simulink model "model_ColumnSetup_00_pre_fable_mux_runtime_retry_20260703_051745"  (R2020b)
settings: Solver=ode4  StartTime=0.0  StopTime=tend  FixedStep=dt  RelTol=1e-3  EnableMultiTasking=on
model workspace (MAT data in the model file):
  controller_enable_switch = Simulink.Parameter
  controller_enable_switch.Value = 0
  controller_enable_switch.DataType = 'boolean'
  controller_enable_switch.Dimensions = [1 1]
  dd_pause_enable = Simulink.Parameter
  dd_pause_enable.Value = 1
  dd_pause_enable.Description = 'Dashboard flag for pausing time-history and sine command generation.'
  dd_pause_enable.DataType = 'auto'
  dd_pause_enable.Dimensions = [1 1]
  osi_gain_enable_initial = Simulink.Parameter
  osi_gain_enable_initial.Value = 0
  osi_gain_enable_initial.DataType = 'auto'
  osi_gain_enable_initial.Dimensions = [1 1]
  smooth_stop_enable = Simulink.Parameter
  smooth_stop_enable.Value = 1
  smooth_stop_enable.Description = 'Dashboard flag for smooth stop and smooth resume of the command.'
  smooth_stop_enable.DataType = 'auto'
  smooth_stop_enable.Dimensions = [1 1]
  zero_meas_enable = Simulink.Parameter
  zero_meas_enable.Value = 0
  zero_meas_enable.Description = 'Dashboard flag for actuator-on adaptive command trim that drives measured displacement back to zero.'
  zero_meas_enable.DataType = 'auto'
  zero_meas_enable.Dimensions = [1 1]
undefined symbols (not defined in the file or in its folder): amp_2_percentile, blwnStdFromExceedance, command_channel_selector, correction_gain, dt, exceed_percentile, f1, f_final, f_init, fbla, fblag, fblbins, fblfbins, fblfw, fbls, fblw, hs_ag, hs_C, hs_force_sign_codegen, hs_force_to_floor, hs_ground_force_gain, hs_interface_from_floor, hs_interface_from_force, hs_K, hs_M, hs_time, hs_time_scale_factor_codegen, phase_lead_den, phase_lead_num, sat_limit, t_ending, tend_chirp, time_history, v2a_gain, v2d_gain, v2f_gain, zero_alpha
libraries: simulink x2, speedgoatlib_IO113 x2, speedgoatlib_IO112 x2, dsparch4 x1, slrealtimeloglib x1, slpidlib x1
settings Model: SimulationMode=external  ExtModeEnableFloating=off  OrderedModelArguments=off  Creator=User  LastModifiedBy=BOWN1111PC1
settings SolverCC: ConcurrentTasks=on  PositivePriorityOrder=on
settings DataIOCC: LimitDataPoints=on  SaveFormat=Array  ReturnWorkspaceOutputs=off
settings OptimizationCC: BlockReduction=off  OptimizeBlockIOStorage=off  BufferReuse=off  ExpressionFolding=off  LocalBlockOutputs=off
settings DebuggingCC: UnderspecifiedInitializationDetection=Classic  MergeDetectMultiDrivingBlocksExec=none  SolverPrmCheckMsg=warning  TasksWithSamePriorityMsg=none  StateNameClashWarn=warning  SFUnexpectedBacktrackingDiag=warning  SFNoUnconditionalDefaultTransitionDiag=warning  SFExecutionAtInitializationDiag=none  ArithmeticOperatorsInVariantConditions=warning
settings HardwareCC: ProdBitPerLong=64  ProdLongLongMode=on  ProdHWDeviceType=Intel->x86-64 (Linux 64)
settings ModelReferenceCC: PropagateSignalLabelsOutOfModel=off
settings SFSimCC: SimUseLocalCustomCode=off  CustomCodeUndefinedFunction=UseInterfaceOnly
settings RTWCC: Description=Simulink Real-Time  SystemTargetFile=slrealtime.tlc  TemplateMakefile=slrealtime_default_tmf  RTWVerbose=off  RTWUseLocalCustomCode=off  Toolchain=Simulink Real-Time Toolchain  BuildConfiguration=Faster Runs  CodeExecutionProfiling=on  TargetLang=C++
settings CodeAppCC: StateflowObjectComments=on
settings ConfigComp: CovMetricSettings=dw  CovSaveCumulativeToWorkspaceVar=on  CovSaveSingleToWorkspaceVar=on  CovExternalEMLEnable=off

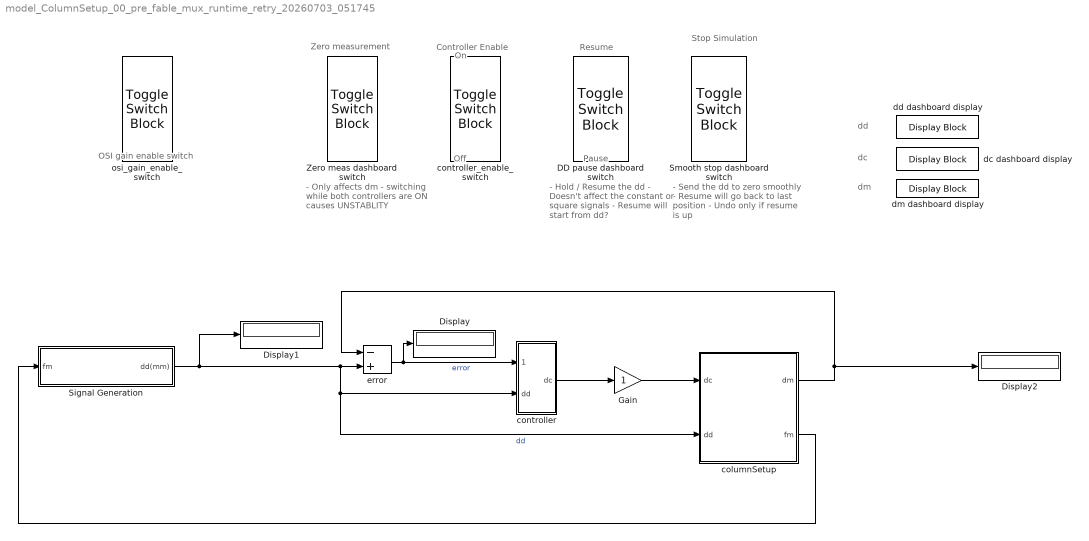
== system model_ColumnSetup_00_pre_fable_mux_runtime_retry_20260703_051745 ==
  note: Pause
  note: Resume
  note: Stop Simulation
  note: - Send the dd to zero smoothly
      | - Resume will go back to last position
      | - Undo only if resume is up
  note: Zero measurement
  note: - Hold / Resume the dd
      | - Doesn't affect the constant or square signals
      | - Resume will start from dd?
  note: - Only affects dm
      | - switching while both controllers are ON causes UNSTABLITY
  note: dd
  note: dc
  note: dm
  note: Controller Enable
  note: On
  note: Off
  note: OSI gain enable switch
  DD pause dashboard switch : ToggleSwitchBlock  LabelPosition=Hide
      settings: Values={{'Zero', ''}, [1 0]}
  Display : Display
      settings: SampleTime=dt
  Display1 : Display
      settings: SampleTime=dt
  Display2 : Display
      settings: SampleTime=dt
  Gain : Gain
  Signal Generation : Subsystem
  Smooth stop dashboard switch : ToggleSwitchBlock  LabelPosition=Hide
      settings: Values={{'Zero', ''}, [0 1]}
  Zero meas dashboard switch : ToggleSwitchBlock  LabelPosition=Hide
      settings: Values={{'Zero', ''}, [0 1]}
  columnSetup : Subsystem
  controller : Subsystem
  controller_enable_switch : ToggleSwitchBlock  LabelPosition=Hide
      settings: Values={{'zero', ''}, [0 1]}
  dc dashboard display : DisplayBlock  LabelPosition=Hide  Format=Custom  Transparency=1  FormatString=%.3f
  dd dashboard display : DisplayBlock  LabelPosition=Hide  Format=Custom  Transparency=1  FormatString=%.3f
  dm dashboard display : DisplayBlock  LabelPosition=Hide  Format=Custom  Transparency=1  FormatString=%.3f
  error : Sum  Inputs=-+  SampleTime=dt
  osi_gain_enable_switch : ToggleSwitchBlock  LabelPosition=Hide
      settings: Values={{'zero', ''}, [0 1]}
  wires:
  columnSetup/1(dm) -> error/1, Display2/1
  error/1 -> Display/1, controller/1(error)  "error"
  controller/1(dc) -> Gain/1
  Signal Generation/1(dd(mm)) -> columnSetup/2(dd), controller/2(dd), error/2, Display1/1  "dd"
  columnSetup/2(fm) -> Signal Generation/1(fm)
  Gain/1 -> columnSetup/1(dc)

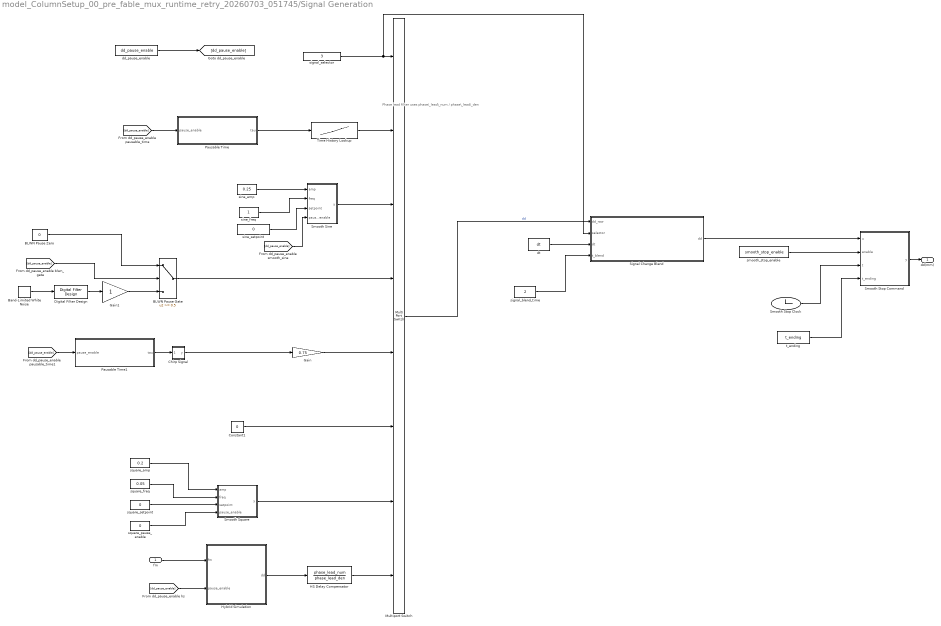
== system model_ColumnSetup_00_pre_fable_mux_runtime_retry_20260703_051745/Signal Generation ==
  note: Phase lead filter uses phase\_lead\_num / phase\_lead\_den
  fm : Inport
  BLWN Pause Gate : Switch  Threshold=0.5  SampleTime=dt
  BLWN Pause Zero : Constant  Value=0  SampleTime=dt
  Band-Limited White Noise : simulink/Sources/Band-Limited White Noise  Cov=blwnStdFromExceedance(amp_2_percentile, exceed_percentile)^2*dt/sum((fir1(130, 2*f1*dt)).^2)  Ts=dt  seed=[22451]
  Chirp Signal : Subsystem  AncestorBlock=simulink/Sources/Chirp Signal  mask(chirp){f1=f_init, T=tend_chirp, f2=f_final, VectorParams1D=on}
      mask prompts: f1 "Simulink:masks:InitialFrequencyHz_MP"; T "Simulink:masks:TargetTimesecs_MP"; f2 "Simulink:masks:FrequencyAtTargetTimeHz_MP"; VectorParams1D "Simulink:masks:InterpretVectorParametersAs1D_MP"
      mask help: Simulink:masks:chirp_MD
      mask init:
      | blkName = gcb;
      | t=[0:.1:5];
      | set_param([blkName '/targetTime'], 'VectorParams1D', VectorParams1D);
      | set_param([blkName '/initialFreq'], 'VectorParams1D', VectorParams1D);
      | set_param([blkName '/deltaFreq'], 'VectorParams1D', VectorParams1D);
      mask Help: The chirp signal has linearly increasing frequency with time.  This block can be used for spectral analysis of nonlinear systems.
      mask Display: plot(t,sin(t.*t))
  Constant1 : Constant  Value=0  SampleTime=dt
  Digital Filter Design : dsparch4/Digital Filter Design  mwdsp_browser_bugfix_var=off
      link override Digital Filter: Coefficients=fir1(130, 2*f1*dt)
  Gain : Gain  Gain=0.75  SampleTime=dt
  Gain1 : Gain  SampleTime=dt
  HS Delay Compensator : DiscreteTransferFcn  Numerator=phase_lead_num  Denominator=phase_lead_den  SampleTime=dt
  Hybrid Simulation : MATLAB Function  TreatAsAtomicUnit=on
  Multiport Switch : MultiPortSwitch  Inputs=7  SampleTime=dt
  Pausable Time : MATLAB Function  TreatAsAtomicUnit=on
  Pausable Time1 : MATLAB Function  TreatAsAtomicUnit=on
  Signal Change Blend : MATLAB Function  TreatAsAtomicUnit=on
  Smooth Sine : MATLAB Function  TreatAsAtomicUnit=on
  Smooth Square : MATLAB Function  TreatAsAtomicUnit=on
  Smooth Stop Clock : Clock
  Smooth Stop Command : MATLAB Function  TreatAsAtomicUnit=on
  Time History Lookup : Lookup_n-D  NumberOfTableDimensions=1  BreakpointsForDimension1=time_history(:,1)  Table=time_history(:,2)  ExtrapMethod=Clip  SampleTime=dt  InternalRulePriority=Speed  RndMeth=Simplest  InputSameDT=on
  dd_pause_enable : Constant  Value=dd_pause_enable  SampleTime=dt
  dt : Constant  Value=dt  SampleTime=dt
  signal_blend_time : Constant  Value=2  SampleTime=dt
  signal_selector : Constant  Value=3  SampleTime=dt
  sine_amp : Constant  Value=0.25  SampleTime=dt
  sine_freq : Constant  SampleTime=dt
  sine_setpoint : Constant  Value=0  SampleTime=dt
  smooth_stop_enable : Constant  Value=smooth_stop_enable  SampleTime=dt
  square_amp : Constant  Value=0.2  SampleTime=dt
  square_freq : Constant  Value=0.05  SampleTime=dt
  square_pause_enable : Constant  Value=0  SampleTime=dt
  square_setpoint : Constant  Value=0  SampleTime=dt
  t_ending : Constant  Value=t_ending  SampleTime=dt
  dd(mm) : Outport  SampleTime=dt
  wires:
  signal_selector/1 -> Signal Change Blend/2(selector), Multiport Switch/1
  Chirp Signal/1(y) -> Gain/1
  Smooth Sine/1(y) -> Multiport Switch/3
  Band-Limited White Noise/1 -> Digital Filter Design/1
  Digital Filter Design/1 -> Gain1/1
  Gain/1 -> Multiport Switch/5
  Constant1/1 -> Multiport Switch/6
  Pausable Time/1(tau) -> Time History Lookup/1
  Time History Lookup/1 -> Multiport Switch/2
  BLWN Pause Zero/1 -> BLWN Pause Gate/1
  Gain1/1 -> BLWN Pause Gate/3
  BLWN Pause Gate/1 -> Multiport Switch/4
  [dd_pause_enable] -> Pausable Time/1(pause_enable)
  [dd_pause_enable] -> BLWN Pause Gate/2
  Pausable Time1/1(tau) -> Chirp Signal/1(tau)
  [dd_pause_enable] -> Pausable Time1/1(pause_enable)
  sine_amp/1 -> Smooth Sine/1(amp)
  sine_freq/1 -> Smooth Sine/2(freq)
  sine_setpoint/1 -> Smooth Sine/3(setpoint)
  [dd_pause_enable] -> Smooth Sine/4(pause_enable)
  smooth_stop_enable/1 -> Smooth Stop Command/2(enable)
  Smooth Stop Clock/1 -> Smooth Stop Command/3(t)
  t_ending/1 -> Smooth Stop Command/4(t_ending)
  dt/1 -> Signal Change Blend/3(dt)
  signal_blend_time/1 -> Signal Change Blend/4(t_blend)
  Multiport Switch/1 -> Signal Change Blend/1(dd_raw)  "dd"
  Signal Change Blend/1(dd) -> Smooth Stop Command/1(u)
  square_amp/1 -> Smooth Square/1(amp)
  square_freq/1 -> Smooth Square/2(freq)
  square_setpoint/1 -> Smooth Square/3(setpoint)
  square_pause_enable/1 -> Smooth Square/4(pause_enable)
  Smooth Square/1(y) -> Multiport Switch/7
  Smooth Stop Command/1(y) -> dd(mm)/1
  dd_pause_enable/1 -> [dd_pause_enable]
  fm/1 -> Hybrid Simulation/1(fm)
  [dd_pause_enable] -> Hybrid Simulation/2(pause_enable)
  Hybrid Simulation/1(dd) -> HS Delay Compensator/1
  HS Delay Compensator/1 -> Multiport Switch/8

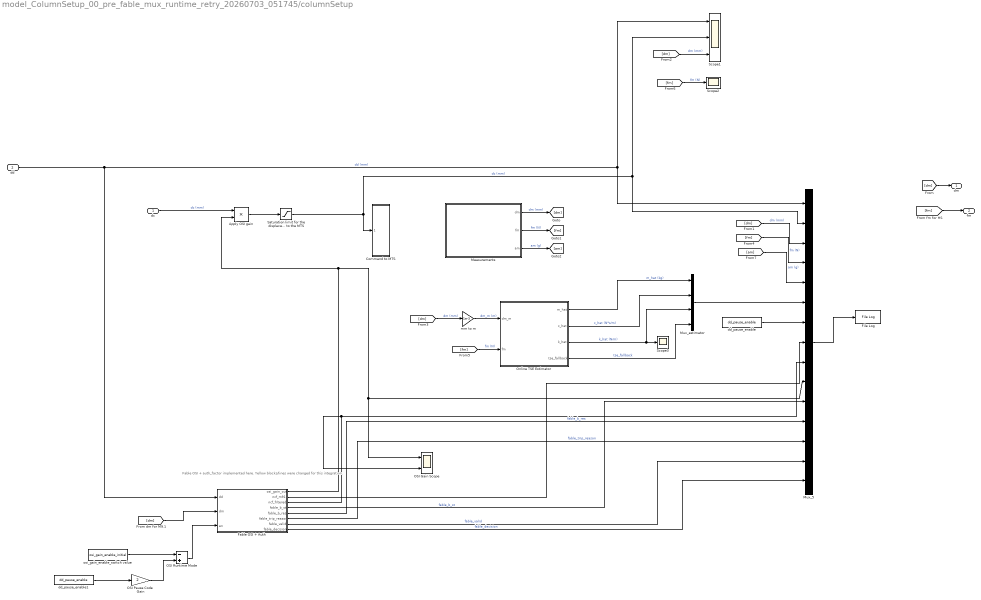
== system model_ColumnSetup_00_pre_fable_mux_runtime_retry_20260703_051745/columnSetup ==
  note: Fable OSI + auth_factor implemented here. Yellow blocks/lines were changed for this integration.
  dc : Inport  SampleTime=dt
  dd : Inport  Port=2  SampleTime=dt
  Apply OSI gain : Product  Inputs=**
  Command to MTS : Subsystem
  Fable OSI + Auth : MATLAB Function  TreatAsAtomicUnit=on
  File Log : slrealtimeloglib/File Log  decimation=1
      settings: SourceProductBaseCode=XP
  Measurements : Subsystem
  Mux_5 : Mux  Inputs=15
  Mux_estimator : Mux
  OSI Gain Scope : Scope  NumInputPorts=2
  OSI Pause Code Gain : Gain  Gain=2
  OSI Runtime Mode : Sum  Inputs=-+  SampleTime=dt
  Online TSE Estimator : MATLAB Function  TreatAsAtomicUnit=on
  Saturation limit for the displacement signal that is sent to the MTS : Saturate  UpperLimit=sat_limit  LowerLimit=-sat_limit  SampleTime=dt
  Scope1 : Scope  NumInputPorts=3
  Scope2 : Scope
  Scope3 : Scope
  dd_pause_enable : Constant  Value=dd_pause_enable  SampleTime=dt
  dd_pause_enable1 : Constant  Value=dd_pause_enable  SampleTime=dt
  mm to m : Gain  Gain=1e-3
  osi_gain_enable_switch value : Constant  Value=osi_gain_enable_initial
  dm : Outport  SampleTime=dt
  fm : Outport  Port=2  SampleTime=dt
  wires:
  Saturation limit for the displacement signal that is sent to the MTS/1 -> Mux_5/2, Scope1/2, Command to MTS/1(dc (mm))  "dc (mm)"
  Mux_5/1 -> File Log/1
  Measurements/1(dm) -> [dm]  "dm (mm)"
  [am] -> Mux_5/5  "am (g)"
  dd/1 -> Mux_5/1, Scope1/1, Fable OSI + Auth/1(dd)  "dd (mm)"
  Online TSE Estimator/1(m_hat) -> Mux_estimator/1  "m_hat (kg)"
  Online TSE Estimator/2(c_hat) -> Mux_estimator/2  "c_hat (N*s/m)"
  Online TSE Estimator/3(k_hat) -> Scope3/1, Mux_estimator/3  "k_hat (N/m)"
  Online TSE Estimator/4(tse_fallback) -> Mux_estimator/4  "tse_fallback"
  [dm] -> dm/1
  [dm] -> Mux_5/3  "dm (mm)"
  [dm] -> Scope1/3  "dm (mm)"
  Measurements/2(fm) -> [fm]  "fm (N)"
  [fm] -> Mux_5/4  "fm (N)"
  [fm] -> Online TSE Estimator/2(fm)  "fm (N)"
  [fm] -> Scope2/1  "fm (N)"
  Measurements/3(am) -> [am]  "am (g)"
  Mux_estimator/1 -> Mux_5/6
  [dm] -> mm to m/1  "dm (mm)"
  mm to m/1 -> Online TSE Estimator/1(dm_m)  "dm_m (m)"
  [fm] -> fm/1
  dd_pause_enable/1 -> Mux_5/7
  dc/1 -> Apply OSI gain/1  "dc (mm)"
  Apply OSI gain/1 -> Saturation limit for the displacement signal that is sent to the MTS/1
  osi_gain_enable_switch value/1 -> OSI Runtime Mode/1
  Fable OSI + Auth/1(osi_gain_out) -> Apply OSI gain/2, OSI Gain Scope/1, Mux_5/10
  Fable OSI + Auth/3(ncf_filtered) -> OSI Gain Scope/2, Mux_5/9
  Fable OSI + Auth/2(ncf_m91) -> Mux_5/8
  [dm] -> Fable OSI + Auth/2(dm)
  OSI Pause Code Gain/1 -> OSI Runtime Mode/2
  OSI Runtime Mode/1 -> Fable OSI + Auth/3(en)
  Fable OSI + Auth/4(fable_b_st) -> Mux_5/11  "fable_b_st"
  Fable OSI + Auth/5(fable_b_res) -> Mux_5/12  "fable_b_res"
  Fable OSI + Auth/6(fable_trip_reason) -> Mux_5/13  "fable_trip_reason"
  Fable OSI + Auth/7(fable_valid) -> Mux_5/14  "fable_valid"
  Fable OSI + Auth/8(fable_decision) -> Mux_5/15  "fable_decision"
  dd_pause_enable1/1 -> OSI Pause Code Gain/1

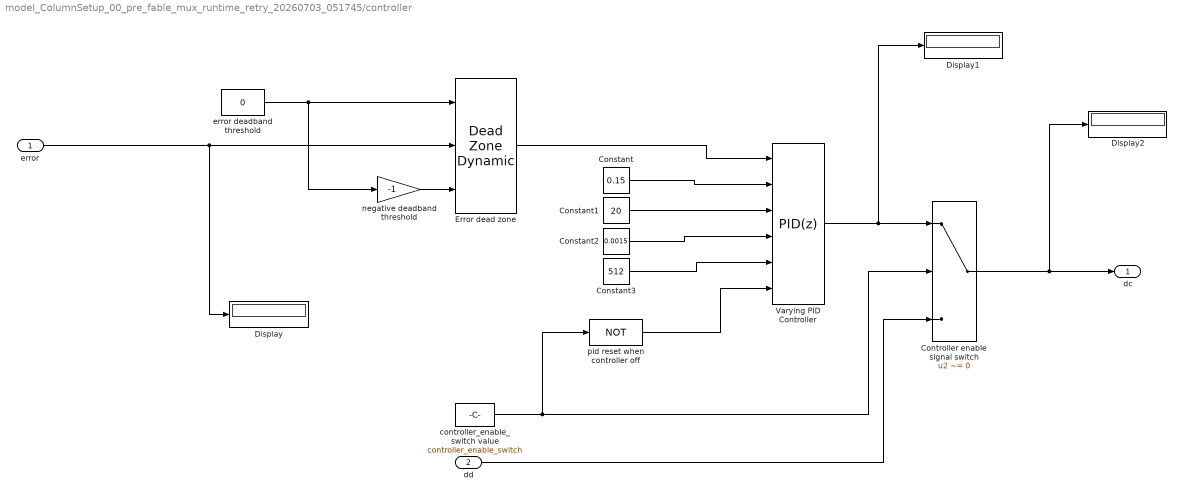
== system model_ColumnSetup_00_pre_fable_mux_runtime_retry_20260703_051745/controller ==
  error : Inport  SampleTime=dt
  dd : Inport  Port=2  SampleTime=dt
  Constant : Constant  Value=0.15  SampleTime=dt
  Constant1 : Constant  Value=20  SampleTime=dt
  Constant2 : Constant  Value=0.0015  SampleTime=dt
  Constant3 : Constant  Value=512  SampleTime=dt
  Controller enable signal switch : Switch  Criteria=u2 ~= 0  SampleTime=dt
  Display : Display
      settings: SampleTime=dt
  Display1 : Display
      settings: SampleTime=dt
  Display2 : Display
      settings: SampleTime=dt
  Error dead zone : simulink/Discontinuities/Dead Zone Dynamic
      settings: SourceProductBaseCode=SL
  Varying PID Controller : slpidlib/PID Controller  Controller=PID  Form=Parallel  TimeDomain=Discrete-time  UseExternalTs=off  SampleTime=dt  IntegratorMethod=Forward Euler  FilterMethod=Forward Euler  ControllerParametersSource=external  P=1  I=1  D=0  UseFilter=on  N=100  TunerSelectOption=Transfer Function Based (PID Tuner App)  InitialConditionSource=internal  InitialConditionForIntegrator=0  InitialConditionForFilter=0  DifferentiatorICPrevScaledInput=0  ExternalReset=level  TrackingMode=off  Kt=1  LimitOutput=off  SatLimitsSource=internal  UpperSaturationLimit=inf  LowerSaturationLimit=-inf  LinearizeAsGain=on  AntiWindupMode=none  Kb=1  POutMin=[]  POutMax=[]  IOutMin=[]  IOutMax=[]  DOutMin=[]  DOutMax=[]  NOutMin=[]  NOutMax=[]  SumOutMin=[]  SumOutMax=[]  SaturationOutMin=[]  SaturationOutMax=[]  PParamMin=[]  PParamMax=[]  IParamMin=[]  IParamMax=[]  DParamMin=[]  DParamMax=[]  NParamMin=[]  NParamMax=[]  KbParamMin=[]  KbParamMax=[]  KtParamMin=[]  KtParamMax=[]  KbOutMin=[]  KbOutMax=[]  KtOutMin=[]  KtOutMax=[]  IntegratorOutMin=[]  IntegratorOutMax=[]  FilterOutMin=[]  FilterOutMax=[]  SumI1OutMin=[]  SumI1OutMax=[]  SumI2OutMin=[]  SumI2OutMax=[]  SumI3OutMin=[]  SumI3OutMax=[]  SumI4OutMin=[]  SumI4OutMax=[]  SumDOutMin=[]  SumDOutMax=[]  DifferentiatorOutMin=[]  DifferentiatorOutMax=[]  FilterDiffOutCoefMin=[]  FilterDiffOutCoefMax=[]  ReciprocalOutMin=[]  ReciprocalOutMax=[]  SumDenOutMin=[]  SumDenOutMax=[]  SumNumOutMin=[]  SumNumOutMax=[]  DivideOutMin=[]  DivideOutMax=[]  UdiffTsProdOutMin=[]  UdiffTsProdOutMax=[]  NTsProdOutMin=[]  NTsProdOutMax=[]  UintegralTsProdOutMin=[]  UintegralTsProdOutMax=[]  UngainTsProdOutMin=[]  UngainTsProdOutMax=[]  IntegratorContinuousStateAttributes=''  IntegratorStateMustResolveToSignalObject=off  IntegratorRTWStateStorageClass=Auto  FilterContinuousStateAttributes=''  FilterStateMustResolveToSignalObject=off  FilterRTWStateStorageClass=Auto  ParallelPVariant=ExternalParameters  IdealPVariant=Disabled  IVariant=ExternalParameters  DVariant=ExternalParameters  IntegratorVariant=Discrete  SatVariant=Disabled  AWVariant=Passthrough  PCopyVariant=Disabled  TRVariant=Disabled  FdbkBlocksVariant=Forward  IdealPFdbkVariant=Disabled  SatFdbkVariant=Disabled  DerivativeFilterVariant=ForwardEulerFilter  NVariant=ExternalParameters  NCopyVariant=Disabled  FilterICVariant=InternalICsFilter  IntegratorICVariant=InternalICs  ExternalResetVariant=ExternalReset  TRSumVariant=Passthrough  SumFdbkVariant=Disabled  SumVariant=Sum_PID  TsampFilterVariant=InternalTs  TsampNgainVariant=Passthrough  TsampIntegralVariant=Passthrough  ExternalSaturationOutDataTypeStr=Inherit: Same as second input
  controller_enable_switch value : Constant  Value=controller_enable_switch  OutDataTypeStr=boolean  SampleTime=dt
  error deadband threshold : Constant  Value=0
  negative deadband threshold : Gain  Gain=-1
  pid reset when controller off : Logic  Operator=NOT  AllPortsSameDT=off  OutDataTypeStr=boolean
  dc : Outport  SampleTime=dt
  wires:
  error/1 -> Error dead zone/2, Display/1
  controller_enable_switch value/1 -> Controller enable signal switch/2, pid reset when controller off/1
  Controller enable signal switch/1 -> Display2/1, dc/1
  Constant3/1 -> Varying PID Controller/5
  Constant1/1 -> Varying PID Controller/3
  dd/1 -> Controller enable signal switch/3
  Constant2/1 -> Varying PID Controller/4
  Constant/1 -> Varying PID Controller/2
  Varying PID Controller/1 -> Display1/1, Controller enable signal switch/1
  pid reset when controller off/1 -> Varying PID Controller/6
  error deadband threshold/1 -> negative deadband threshold/1, Error dead zone/1
  negative deadband threshold/1 -> Error dead zone/3
  Error dead zone/1 -> Varying PID Controller/1

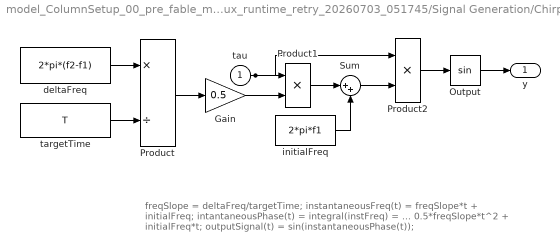
== system model_ColumnSetup_00_pre_fable_mux_runtime_retry_20260703_051745/Signal Generation/Chirp Signal ==
  note: freqSlope = deltaFreq/targetTime;
      | instantaneousFreq(t) = freqSlope*t + initialFreq;
      | intantaneousPhase(t) = integral(instFreq) = ...
      |       0.5*freqSlope*t^2 + initialFreq*t;
      | outputSignal(t) = sin(instantaneousPhase(t));
  tau : Inport
  Gain : Gain  DisableCoverage=on  Gain=0.5  OutDataTypeStr=Inherit: Same as input  ParamDataTypeStr=Inherit: Same as input
  Output : Trigonometry
  Product : Product  DisableCoverage=on  Inputs=*/  InputSameDT=on  SaturateOnIntegerOverflow=on  OutDataTypeStr=Inherit: Same as first input
  Product1 : Product  DisableCoverage=on  InputSameDT=on  SaturateOnIntegerOverflow=on  OutDataTypeStr=Inherit: Same as first input
  Product2 : Product  DisableCoverage=on  InputSameDT=on  SaturateOnIntegerOverflow=on  OutDataTypeStr=Inherit: Same as first input
  Sum : Sum  DisableCoverage=on  Inputs=|++  InputSameDT=on  SaturateOnIntegerOverflow=on  OutDataTypeStr=Inherit: Same as first input
  deltaFreq : Constant  DisableCoverage=on  Value=2*pi*(f2-f1)
  initialFreq : Constant  DisableCoverage=on  Value=2*pi*f1
  targetTime : Constant  DisableCoverage=on  Value=T
  y : Outport
  wires:
  Output/1 -> y/1
  Product2/1 -> Output/1
  Sum/1 -> Product2/2
  initialFreq/1 -> Sum/2
  Product1/1 -> Sum/1
  Gain/1 -> Product1/2
  Product/1 -> Gain/1
  targetTime/1 -> Product/2
  deltaFreq/1 -> Product/1
  tau/1 -> Product2/1, Product1/1

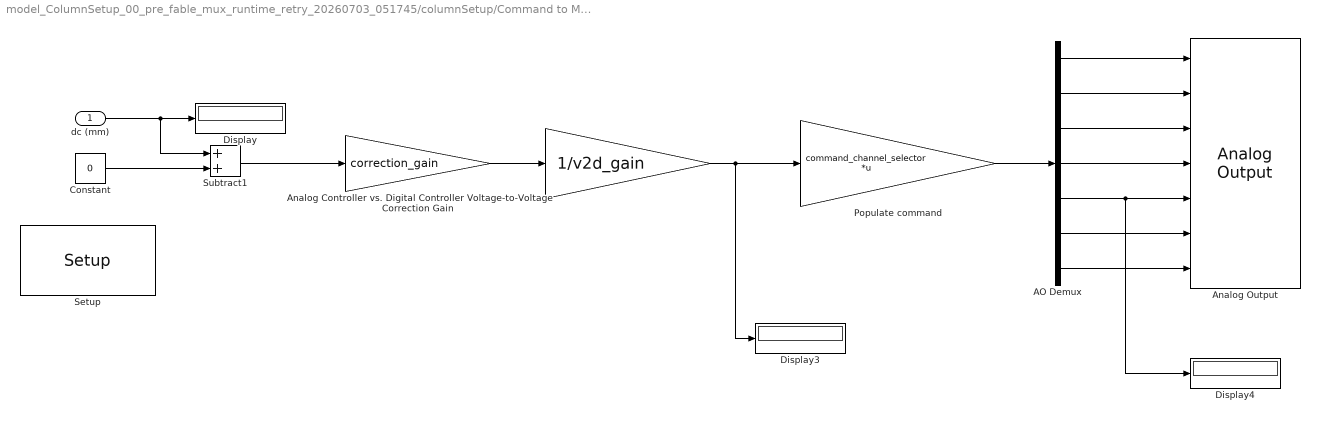
== system model_ColumnSetup_00_pre_fable_mux_runtime_retry_20260703_051745/columnSetup/Command to MTS ==
  dc (mm) : Inport  SampleTime=dt
  "  " : Gain  Gain=1/v2d_gain  SampleTime=dt
  " Analog Controller vs. Digital Controller Voltage-to-Voltage Correction Gain  " : Gain  Gain=correction_gain  SampleTime=dt
  AO Demux : Demux  Outputs=7
  Analog Output : speedgoatlib_IO113/Analog Output  id=1  index=[1,2,3,4,5,6,7]  channels=[1,2,3,4,5,6,7]  range=1  ts=dt  pciSlot=-1
      settings: SourceProductName=Simulink Real-Time: Speedgoat I/O Blockset
  Constant : Constant  Value=0  SampleTime=dt
  Display : Display
      settings: SampleTime=dt
  Display3 : Display
      settings: SampleTime=dt
  Display4 : Display
      settings: SampleTime=dt
  Populate command : Gain  Gain=command_channel_selector  Multiplication=Matrix(K*u)  SampleTime=dt
  Setup : speedgoatlib_IO113/Setup  group=Analog output setup  id=1  range=+-10V  daMode=Differential  triggerSignal=TTL  cal=off  dioDirLo=Output  dioDirHi=Input  pciSlot=-1  daChannel=[1,2,3,4,5,6,7]  daInitValue=[0 0 0 0 0 0 0]  daReset=[0]  doChannel=[1,2,3,4]  diChannel=[5,6,7,8]  doInitValue=[0]  doReset=[1]
      settings: SourceProductName=Simulink Real-Time: Speedgoat I/O Blockset
  Subtract1 : Sum  SampleTime=dt
  wires:
  " Analog Controller vs. Digital Controller Voltage-to-Voltage Correction Gain  "/1 -> "  "/1
  AO Demux/6 -> Analog Output/6
  AO Demux/3 -> Analog Output/3
  AO Demux/1 -> Analog Output/1
  AO Demux/4 -> Analog Output/4
  AO Demux/2 -> Analog Output/2
  Constant/1 -> Subtract1/2
  AO Demux/7 -> Analog Output/7
  Populate command/1 -> AO Demux/1
  Subtract1/1 -> " Analog Controller vs. Digital Controller Voltage-to-Voltage Correction Gain  "/1
  "  "/1 -> Display3/1, Populate command/1
  dc (mm)/1 -> Subtract1/1, Display/1
  AO Demux/5 -> Display4/1, Analog Output/5

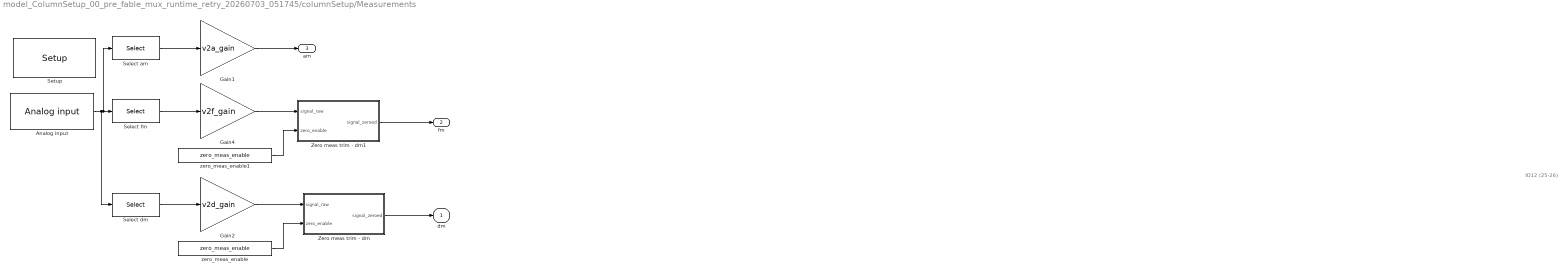
== system model_ColumnSetup_00_pre_fable_mux_runtime_retry_20260703_051745/columnSetup/Measurements ==
  note: IO12 (25-26)
  Analog input : speedgoatlib_IO112/Analog input  id=1  ts=dt  channels=18  range=1  resolution=1  pciSlot=-1
      settings: SourceProductName=Simulink Real-Time: Speedgoat I/O Blockset
  Gain1 : Gain  Gain=v2a_gain  SampleTime=dt
  Gain2 : Gain  Gain=v2d_gain  SampleTime=dt
  Gain4 : Gain  Gain=v2f_gain  SampleTime=dt
  Select am : Selector  InputPortWidth=18  SampleTime=dt  IndexOptions=Index vector (dialog)  Indices=ch.am  OutputSizes=1
  Select dm : Selector  InputPortWidth=18  SampleTime=dt  IndexOptions=Index vector (dialog)  Indices=ch.dm  OutputSizes=1
  Select fm : Selector  InputPortWidth=18  SampleTime=dt  IndexOptions=Index vector (dialog)  Indices=ch.fm  OutputSizes=1
  Setup : speedgoatlib_IO112/Setup  group=Analog input setup  id=1  cal=off  initiator=Initiator  invertIO=off  pciSlot=-1  adResolution=18bit (no data packing)  adChannel=18  adRange=+-10V  adCoupling=Differential
      settings: SourceProductName=Simulink Real-Time: Speedgoat I/O Blockset
  Zero meas trim - dm : Subsystem
  Zero meas trim - dm1 : Subsystem
  zero_meas_enable : Constant  Value=zero_meas_enable  SampleTime=dt
  zero_meas_enable1 : Constant  Value=zero_meas_enable  SampleTime=dt
  dm : Outport  SampleTime=dt
  fm : Outport  Port=2  SampleTime=dt
  am : Outport  Port=3  SampleTime=dt
  wires:
  Gain2/1 -> Zero meas trim - dm/1(signal_raw)
  Gain4/1 -> Zero meas trim - dm1/1(signal_raw)
  zero_meas_enable1/1 -> Zero meas trim - dm1/2(zero_enable)
  zero_meas_enable/1 -> Zero meas trim - dm/2(zero_enable)
  Zero meas trim - dm1/1(signal_zeroed) -> fm/1
  Zero meas trim - dm/1(signal_zeroed) -> dm/1
  Select dm/1 -> Gain2/1
  Select am/1 -> Gain1/1
  Select fm/1 -> Gain4/1
  Gain1/1 -> am/1
  Analog input/1 -> Select fm/1, Select am/1, Select dm/1

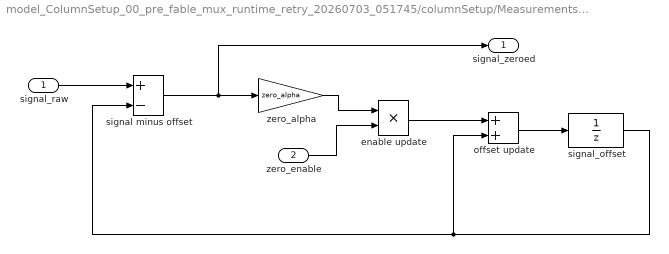
== system model_ColumnSetup_00_pre_fable_mux_runtime_retry_20260703_051745/columnSetup/Measurements/Zero meas trim - dm ==
  signal_raw : Inport  SampleTime=dt
  zero_enable : Inport  Port=2  SampleTime=dt
  enable update : Product  SampleTime=dt
  offset update : Sum  SampleTime=dt
  signal minus offset : Sum  Inputs=+-  SampleTime=dt
  signal_offset : UnitDelay  SampleTime=dt  HasFrameUpgradeWarning=on
  zero_alpha : Gain  Gain=zero_alpha  SampleTime=dt
  signal_zeroed : Outport  SampleTime=dt
  wires:
  offset update/1 -> signal_offset/1
  enable update/1 -> offset update/1
  zero_enable/1 -> enable update/2
  zero_alpha/1 -> enable update/1
  signal minus offset/1 -> zero_alpha/1, signal_zeroed/1
  signal_offset/1 -> signal minus offset/2, offset update/2
  signal_raw/1 -> signal minus offset/1

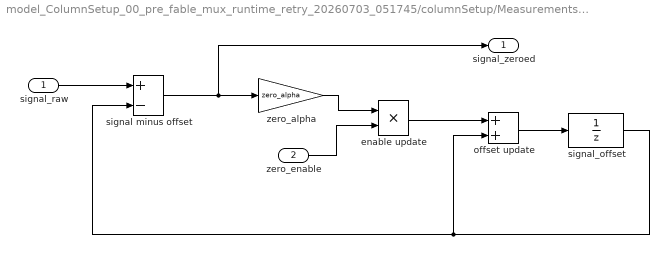
== system model_ColumnSetup_00_pre_fable_mux_runtime_retry_20260703_051745/columnSetup/Measurements/Zero meas trim - dm1 ==
  signal_raw : Inport  SampleTime=dt
  zero_enable : Inport  Port=2  SampleTime=dt
  enable update : Product  SampleTime=dt
  offset update : Sum  SampleTime=dt
  signal minus offset : Sum  Inputs=+-  SampleTime=dt
  signal_offset : UnitDelay  SampleTime=dt  HasFrameUpgradeWarning=on
  zero_alpha : Gain  Gain=zero_alpha  SampleTime=dt
  signal_zeroed : Outport  SampleTime=dt
  wires:
  offset update/1 -> signal_offset/1
  enable update/1 -> offset update/1
  zero_enable/1 -> enable update/2
  zero_alpha/1 -> enable update/1
  signal minus offset/1 -> zero_alpha/1, signal_zeroed/1
  signal_offset/1 -> signal minus offset/2, offset update/2
  signal_raw/1 -> signal minus offset/1

== matlab function model_ColumnSetup_00_pre_fable_mux_runtime_retry_20260703_051745/Signal Generation/Hybrid Simulation ==
  data: fm input; dd output; pause_enable input; hs_M parameter; hs_C parameter; hs_K parameter; hs_force_to_floor parameter; hs_interface_from_floor parameter; hs_interface_from_force parameter; hs_ground_force_gain parameter; hs_time parameter; hs_ag parameter; hs_time_scale_factor_codegen parameter; hs_force_sign_codegen parameter; dt parameter
function dd = hybrid_simulation(fm, pause_enable, hs_M, hs_C, hs_K, hs_force_to_floor, hs_interface_from_floor, hs_interface_from_force, hs_ground_force_gain, hs_time, hs_ag, hs_time_scale_factor_codegen, hs_force_sign_codegen, dt)
%#codegen
% WARNING - SAFETY CRITICAL: this block sends live HS command displacement.
% Keep force sign, interface equations, units, and stepping aligned with step_HS.m and num_exp.m.
persistent state
if isempty(state)
    state = zeros(12, 1);
end
cfg.n_floor = 3;
cfg.M = hs_M;
cfg.C = hs_C;
cfg.K = hs_K;
cfg.force_to_floor = hs_force_to_floor;
cfg.interface_from_floor = hs_interface_from_floor;
cfg.interface_from_force = hs_interface_from_force;
cfg.ground_force_gain = hs_ground_force_gain;
cfg.time = hs_time;
cfg.ag = hs_ag;
cfg.time_scale_factor = hs_time_scale_factor_codegen;
cfg.force_sign = hs_force_sign_codegen;
[dd, state] = step_HS(fm, pause_enable, dt, cfg, state);
end

== matlab function model_ColumnSetup_00_pre_fable_mux_runtime_retry_20260703_051745/columnSetup/Fable OSI + Auth ==
  data: dd input double size=1; osi_gain_out output double size=1; dm input double size=1; en input size=1; ncf_m91 output double size=1; ncf_filtered output double size=1; fable_b_st output; fable_b_res output; fable_trip_reason output; fable_valid output; fable_decision output; fbls parameter; fblw parameter; fblbins parameter; fblfw parameter; fblfbins parameter; fblag parameter; fbla parameter
function [osi_gain_out,ncf_m91,ncf_filtered,fable_b_st,fable_b_res,fable_trip_reason,fable_valid,fable_decision]=fable_osi_update(dd,dm,en,fbls,fblw,fblbins,fblfw,fblfbins,fblag,fbla)
%#codegen
[osi_gain_out,ncf_m91,fable_b_st,fable_b_res,ncf_filtered,fable_trip_reason,fable_valid,fable_decision]=fable_osi_runtime( ...
    dd,dm,en,fbls,fblw,fblbins,fblfw,fblfbins,fblag,fbla);
end

== matlab function model_ColumnSetup_00_pre_fable_mux_runtime_retry_20260703_051745/Signal Generation/Pausable Time ==
  data: pause_enable input; tau output; dt parameter
function tau = pausable_time(pause_enable, dt)
%#codegen
% Units: pause_enable is dimensionless; dt and tau are s.
persistent tau_state
if isempty(tau_state)
    tau_state = 0.0;
end

if pause_enable == 0
    tau_state = tau_state + dt;
end

tau = tau_state;

== matlab function model_ColumnSetup_00_pre_fable_mux_runtime_retry_20260703_051745/Signal Generation/Smooth Sine ==
  data: amp input; y output; freq input; setpoint input; pause_enable input; dt parameter
function y = smooth_sine(amp, freq, setpoint, pause_enable, dt)
%#codegen
% Units: amplitude, setpoint, internal state, and output are mm;
% frequency is Hz; pause flag is dimensionless; dt is s.
persistent phase offset y_prev amp_prev setpoint_prev startup_t startup_y0 startup_active startup_done
if isempty(phase)
    phase = 0.0;
    offset = 0.0;
    y_prev = 0.0;
    amp_prev = amp;
    setpoint_prev = setpoint;
    startup_t = 0.0;
    startup_y0 = 0.0;
    startup_active = false;
    startup_done = false;
end

startup_time = 2.0;

if pause_enable ~= 0
    y = y_prev;
    return
end

if ~startup_done
    if ~startup_active
        startup_active = true;
        startup_t = 0.0;
        startup_y0 = y_prev;
        phase = 0.0;
        offset = 0.0;
    end

    startup_t = min(startup_t + dt, startup_time);
    u = startup_t/startup_time;
    s = u*u*(3.0 - 2.0*u);
    y = startup_y0 + (setpoint - startup_y0)*s;
    y_prev = y;

    if startup_t >= startup_time
        startup_done = true;
        amp_prev = amp;
        setpoint_prev = setpoint;
    end
    return
end

phase = mod(phase + 2.0*pi*freq*dt, 2.0*pi);
raw = setpoint + amp*sin(phase);

if amp ~= amp_prev || setpoint ~= setpoint_prev
    offset = y_prev - raw;
    amp_prev = amp;
    setpoint_prev = setpoint;
end

y = raw + offset;
offset = offset*exp(-dt/0.1);
y_prev = y;

== matlab function model_ColumnSetup_00_pre_fable_mux_runtime_retry_20260703_051745/Signal Generation/Pausable Time1 ==
  data: pause_enable input; tau output; dt parameter
function tau = pausable_time(pause_enable, dt)
%#codegen
% Units: pause_enable is dimensionless; dt and tau are s.
persistent tau_state
if isempty(tau_state)
    tau_state = 0.0;
end

if pause_enable == 0
    tau_state = tau_state + dt;
end

tau = tau_state;

== matlab function model_ColumnSetup_00_pre_fable_mux_runtime_retry_20260703_051745/Signal Generation/Smooth Stop Command ==
  settings: updateMethod=DISCRETE  sampleTime=dt
  data: u input; y output; enable input; t input; t_ending input
function y = smooth_stop_command(u, enable, t, t_ending)
%#codegen
% Units: input/output displacement are mm; enable is dimensionless; times are s.
persistent last_enable t0 blend0 blend
if isempty(last_enable)
    last_enable = false;
    t0 = 0;
    blend0 = 0;
    blend = 0;
end

enable = enable ~= 0;
if enable ~= last_enable
    t0 = t;
    blend0 = blend;
end

target = double(enable);
tau = min(max((t - t0) / max(t_ending, eps), 0), 1);
s = 3*tau^2 - 2*tau^3;
blend = blend0 + (target - blend0)*s;
y = (1 - blend)*u;
last_enable = enable;

== matlab function model_ColumnSetup_00_pre_fable_mux_runtime_retry_20260703_051745/Signal Generation/Smooth Square ==
  data: amp input; y output; freq input; setpoint input; pause_enable input; dt parameter
function y = smooth_square(amp, freq, setpoint, pause_enable, dt)
%#codegen
% Units: amplitude, setpoint, internal state, and output are mm;
% frequency is Hz; pause flag is dimensionless; dt is s.
persistent phase offset y_prev amp_prev setpoint_prev startup_t startup_y0 startup_active startup_done
if isempty(phase)
    phase = 0.0;
    offset = 0.0;
    y_prev = 0.0;
    amp_prev = amp;
    setpoint_prev = setpoint;
    startup_t = 0.0;
    startup_y0 = 0.0;
    startup_active = false;
    startup_done = false;
end

startup_time = 2.0;

if pause_enable ~= 0
    y = y_prev;
    return
end

if ~startup_done
    if ~startup_active
        startup_active = true;
        startup_t = 0.0;
        startup_y0 = y_prev;
        phase = 0.0;
        offset = 0.0;
    end

    startup_t = min(startup_t + dt, startup_time);
    u = startup_t/startup_time;
    s = u*u*(3.0 - 2.0*u);
    y = startup_y0 + (setpoint - startup_y0)*s;
    y_prev = y;

    if startup_t >= startup_time
        startup_done = true;
        amp_prev = amp;
        setpoint_prev = setpoint;
    end
    return
end

phase = mod(phase + freq*dt, 1.0);
if phase < 0.5
    raw = setpoint + amp;
else
    raw = setpoint - amp;
end

if amp ~= amp_prev || setpoint ~= setpoint_prev
    offset = y_prev - raw;
    amp_prev = amp;
    setpoint_prev = setpoint;
end

y = raw + offset;
offset = offset*exp(-dt/0.1);
y_prev = y;

== matlab function model_ColumnSetup_00_pre_fable_mux_runtime_retry_20260703_051745/columnSetup/Online TSE Estimator ==
  data: dm_m input; m_hat output; fm input; c_hat output; k_hat output; tse_fallback output
function [m_hat, c_hat, k_hat, tse_fallback] = online_tse_estimator(dm_m, fm)
%#codegen
% Units: dm_m input is m and fm input is N. m_hat is kg, c_hat is
% N*s/m, k_hat is N/m, and tse_fallback is dimensionless.
% m_hat: online specimen mass estimate [kg].
% c_hat: online specimen damping estimate [N*s/m].
% k_hat: online specimen stiffness estimate [N/m].
% tse_fallback: 0 means the last update accepted TSE; 1 means TSE was not used and the block is using fallback/hold behavior.

    persistent z_buffer sum_z sum_zz sample_index sample_count update_count
    persistent theta_last fallback_last dm_prev v_prev initialized

    dt = 1 / 2048;
    window_samples = 2048;
    update_samples = 64;
    f_min = 120;
    route_ratio_max = 3;
    theta0 = [2.04; 12; 7028000];
    theta_min = 0.02 * theta0;

    if isempty(initialized)
        z_buffer = zeros(2048, 4);
        sum_z = zeros(1, 4);
        sum_zz = zeros(4, 4);
        sample_index = 1;
        sample_count = 0;
        update_count = 0;
        theta_last = theta0;
        fallback_last = true;
        dm_prev = dm_m;
        v_prev = 0;
        initialized = true;
    end

    v = (dm_m - dm_prev) / dt;
    a = (v - v_prev) / dt;
    dm_prev = dm_m;
    v_prev = v;

    z = [a, v, dm_m, fm];
    old = z_buffer(sample_index, :);
    z_buffer(sample_index, :) = z;
    sum_z = sum_z + z - old;
    sum_zz = sum_zz + z.' * z - old.' * old;

    sample_index = sample_index + 1;
    if sample_index > window_samples
        sample_index = 1;
    end
    if sample_count < window_samples
        sample_count = sample_count + 1;
    end

    if sample_count >= window_samples
        update_count = update_count + 1;
        if update_count >= update_samples
            update_count = 0;
            C = sum_zz - (sum_z.' * sum_z) / window_samples;
            C = 0.5 * (C + C.');
            G = C(1:3, 1:3);
            b = C(1:3, 4);
            FF = C(4, 4);
            F_rms = sqrt(max(FF, 0) / window_samples);

            if F_rms <= f_min
                fallback_last = true;
            else
                theta_lse = pinv(G) * b;
                [U, S, V] = svd(C);
                U = U + 0;
                S = S + 0;
                q = V(:, 4);

                if abs(q(4)) > eps
                    theta = -q(1:3) / q(4);
                    sse_lse = max(FF - theta_lse.' * b, 0);
                    sse_tls = max(theta.' * G * theta - 2 * theta.' * b + FF, 0);
                    residual_ratio = sqrt(sse_tls / max(sse_lse, eps));
                    if residual_ratio <= route_ratio_max
                        fallback_last = false;
                    else
                        theta = theta_lse;
                        fallback_last = true;
                    end
                else
                    theta = theta_lse;
                    fallback_last = true;
                end

                if all(isfinite(theta))
                    theta = max(theta, theta_min);
                    theta_last = theta;
                else
                    fallback_last = true;
                end
            end
        end
    end

    m_hat = theta_last(1);
    c_hat = theta_last(2);
    k_hat = theta_last(3);
    tse_fallback = double(fallback_last);
end

== matlab function model_ColumnSetup_00_pre_fable_mux_runtime_retry_20260703_051745/Signal Generation/Signal Change Blend ==
  data: dd_raw input; dd output; selector input; dt input; t_blend input
function dd = signal_change_blend(dd_raw, selector, dt, t_blend)
%#codegen
% Units: dd_raw, internal displacement state, and dd are mm; selector
% is dimensionless; times are s.
persistent selector_prev y_prev y0 blend_t blending
if isempty(selector_prev)
    selector_prev = selector;
    y_prev = dd_raw;
    y0 = dd_raw;
    blend_t = t_blend;
    blending = false;
end

if selector ~= selector_prev
    selector_prev = selector;
    y0 = y_prev;
    blend_t = 0.0;
    blending = true;
end

if blending
    blend_t = min(blend_t + dt, t_blend);
    if t_blend > 0
        u = blend_t/t_blend;
    else
        u = 1.0;
    end
    s = u*u*(3.0 - 2.0*u);
    dd = y0 + s*(dd_raw - y0);
    if blend_t >= t_blend
        blending = false;
    end
else
    dd = dd_raw;
end

y_prev = dd;
